simulink model "ev_battery_sim"  (R2026b)
settings: Solver=ode23t  StopTime=60.0  MaxStep=0.05
undefined symbols (not defined in the file or in its folder): Current_A, Temp_C, Voltage_V
libraries: fl_lib x10, nesl_utility x6, EdgeImpulse_Library x2, batteryecm_lib x1
settings Model: Creator=HP  LastModifiedBy=HP
settings SimscapeCC: SimscapeLogType=all  SimscapeNominalValues="[{\"value\":\"1\",\"unit\":\"A\"},{\"value\":\"1\",\"unit\":\"bar\"},{\"value\":\"1\",\"unit\":\"cm^2\"},{\"value\":\"1\",\"unit\":\"cm^3/s\"},{\"value\":\"1\",\"unit\":\"kJ/kg\"},{\"value\":\"1\",\"unit\":\"kW\"},{\"value\":\"1\",\"unit\":\"l\"},{\"value\":\"1\",\"unit\":\"N\"},{\"value\":\"1\",\"unit\":\"N*m\"},{\"value\":\"1\",\"unit\":\"V\"},{\"value\":\"0.001\",\"unit\":\"Wb\"}]"  SimscapeUseEnergyAccounting=off

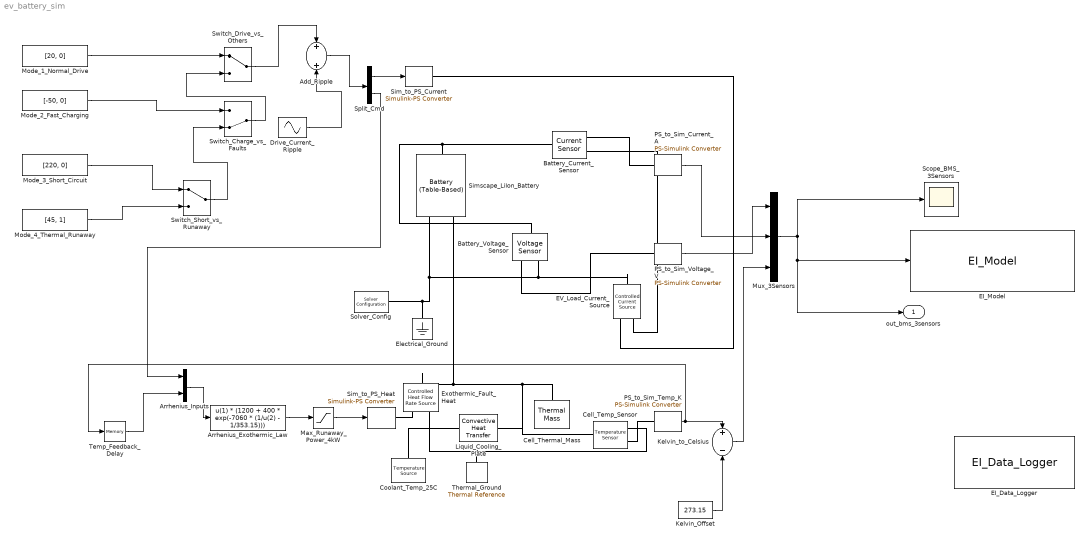
== system ev_battery_sim ==
  Add_Ripple : Sum
  Arrhenius_Exothermic_Law : Fcn  Expr=u(1) * (1200 + 400 * exp(-7060 * (1/u(2) - 1/353.15)))
  Arrhenius_Inputs : Mux  Inputs=2
  Battery_Current_Sensor : fl_lib/Electrical/Electrical Sensors/Current Sensor
  Battery_Voltage_Sensor : fl_lib/Electrical/Electrical Sensors/Voltage Sensor
  Cell_Temp_Sensor : fl_lib/Thermal/Thermal Sensors/Temperature Sensor  temperature_measure=foundation.enum.MeasurementReference.difference
  Cell_Thermal_Mass : fl_lib/Thermal/Thermal Elements/Thermal Mass  mass_type=foundation.enum.constant_variable.constant  mass=0.40 kg  sp_heat=1000 J/(K*kg)  mass_min=1e-6 kg  num_ports=foundation.enum.numPorts2.one  m_specify=off  m_priority=High  m=1 kg  m_nominal_specify=off  m_nominal_value=1  m_nominal_unit=kg  T_specify=on  T_priority=High  T=298.15 K  T_nominal_specify=off  T_nominal_value=1  T_nominal_unit=K  Q_specify=off  Q_priority=None  Q=0 W  Q_nominal_specify=off  Q_nominal_value=1  Q_nominal_unit=W
  Coolant_Temp_25C : fl_lib/Thermal/Thermal Sources/Temperature Source  temperature=298.15 K
  Drive_Current_Ripple : Sin  Amplitude=[2.5, 0]  Frequency=2*pi*0.5  SampleTime=0.05
  EI_Data_Logger : EdgeImpulse_Library/EI_Data_Logger  ei_enabled=on  ei_skip_zero=on  ei_label=Normal_Drive  ei_window_sec=3  ei_max_chunks=0  ei_category=training  ei_sensors=Voltage_V,Current_A,Temp_C  ei_units=V,A,Cel  ei_apikey=ei_bdf74ae27c7bb8ce14bbbb5e7690b771b2b0dc35a7d65027  ei_outdir=default
      settings: SourceProductName=Edge Impulse TinyML
  EI_Model : EdgeImpulse_Library/EI_Model  ei_zip_path=C:\Users\HP\Downloads\bms_system-cpp-mcu-v1-impulse-#1.zip  ei_show_hud=on  ei_verbose=on  ei_step_sec=0.25
      settings: SourceProductName=Edge Impulse TinyML
  EV_Load_Current_Source : fl_lib/Electrical/Electrical Sources/Controlled Current Source
  Electrical_Ground : fl_lib/Electrical/Electrical Elements/Electrical Reference
  Exothermic_Fault_Heat : fl_lib/Thermal/Thermal Sources/Controlled Heat Flow Rate Source
  Kelvin_Offset : Constant  Value=273.15
  Kelvin_to_Celsius : Sum  Inputs=+-
  Liquid_Cooling_Plate : fl_lib/Thermal/Thermal Elements/Convective Heat Transfer  thermal_type=foundation.enum.constant_variable.constant  area=0.02 m^2  heat_tr_coeff=200 W/(K*m^2)  min_heat_tr_coeff=1e-3 W/(K*m^2)  T_specify=off  T_priority=None  T=0 K  T_nominal_specify=off  T_nominal_value=1  T_nominal_unit=K  Q_specify=off  Q_priority=None  Q=0 W  Q_nominal_specify=off  Q_nominal_value=1  Q_nominal_unit=W
  Max_Runaway_Power_4kW : Saturate  UpperLimit=4000  LowerLimit=0
  Mode_1_Normal_Drive : Constant  Value=[20, 0]
  Mode_2_Fast_Charging : Constant  Value=[-50, 0]
  Mode_3_Short_Circuit : Constant  Value=[220, 0]
  Mode_4_Thermal_Runaway : Constant  Value=[45, 1]
  Mux_3Sensors : Mux  Inputs=3
  PS_to_Sim_Current_A : nesl_utility/PS-Simulink Converter  PhysicalDomain=network_engine_domain  SubClassName=ps_output  LeftPortType=input  RightPortType=output  PseudoPeriodic=off  Frequencies=[]  VectorFormat=inherit  Unit=inherit  AffineConversion=off
  PS_to_Sim_Temp_K : nesl_utility/PS-Simulink Converter  PhysicalDomain=network_engine_domain  SubClassName=ps_output  LeftPortType=input  RightPortType=output  PseudoPeriodic=off  Frequencies=[]  VectorFormat=inherit  Unit=inherit  AffineConversion=off
  PS_to_Sim_Voltage_V : nesl_utility/PS-Simulink Converter  PhysicalDomain=network_engine_domain  SubClassName=ps_output  LeftPortType=input  RightPortType=output  PseudoPeriodic=off  Frequencies=[]  VectorFormat=inherit  Unit=inherit  AffineConversion=off
  Scope_BMS_3Sensors : Scope
  Sim_to_PS_Current : nesl_utility/Simulink-PS Converter  PhysicalDomain=network_engine_domain  SubClassName=ps_input  LeftPortType=input  RightPortType=output  PseudoPeriodic=off  Frequencies=[]  NoiseDistribution=none  NoiseParameters=[]  Unit=1  AffineConversion=off  FilteringAndDerivatives=provide  SimscapeFilterOrder=1  InputFilterTimeConstant=0.001  UdotUserProvided=0
  Sim_to_PS_Heat : nesl_utility/Simulink-PS Converter  PhysicalDomain=network_engine_domain  SubClassName=ps_input  LeftPortType=input  RightPortType=output  PseudoPeriodic=off  Frequencies=[]  NoiseDistribution=none  NoiseParameters=[]  Unit=1  AffineConversion=off  FilteringAndDerivatives=provide  SimscapeFilterOrder=1  InputFilterTimeConstant=0.001  UdotUserProvided=0
  Simscape_LiIon_Battery : batteryecm_lib/Battery (Table-Based)  SOC_vec=[0, .1, .25, .5, .75, .9, 1]  T_dependence=simscape.enum.tablebattery.temperature_dependence.yes  prm_dir=simscape.enum.tablebattery.prm_dir.noCurrentDirectionality  T_vec=[278, 293, 313] K  V0_mat=[3.49, 3.5, 3.51; 3.55, 3.57, 3.56; 3.62, 3.63, 3.64; 3.71, 3.71, 3.72; 3.91, 3.93, 3.94; 4.07, 4.08, 4.08; 4.19, 4.19, 4.19] V  V0_vec=[3.5057, 3.566, 3.6337, 3.7127, 3.9259, 4.0777, 4.1928] V  V_range=[0, inf] V  R0_mat=[.0117, .0085, .009; .011, .0085, .009; .0114, .0087, .0092; .0107, .0082, .0088; .0107, .0083, .0091; .0113, .0085, .0089; .0116, .0085, .0089] Ohm  R0_vec=[.0085, .0085, .0087, .0082, .0083, .0085, .0085] Ohm  R0_dis_mat=[.0117, .0085, .009; .011, .0085, .009; .0114, .0087, .0092; .0107, .0082, .0088; .0107, .0083, .0091; .0113, .0085, .0089; .0116, .0085, .0089] Ohm  R0_dis_vec=[.0085, .0085, .0087, .0082, .0083, .0085, .0085] Ohm  R0_ch_mat=[.0117, .0085, .009; .011, .0085, .009; .0114, .0087, .0092; .0107, .0082, .0088; .0107, .0083, .0091; .0113, .0085, .0089; .0116, .0085, .0089] Ohm  R0_ch_vec=[.0085, .0085, .0087, .0082, .0083, .0085, .0085] Ohm  AH=27 A*hr  prm_leak=simscape.enum.tablebattery.prm_leak.disabled  Rleak_vec=[8000, 7000, 6000] Ohm  Rleak=7e3 Ohm  extrapolation_option=simscape.enum.extrapolation.nearest  SOC_port=simscape.enum.tablebattery.enable.no  prm_dyn=simscape.enum.tablebattery.prm_dyn.off  R1_mat=[.0109, .0029, .0013; .0069, .0024, .0012; .0047, .0026, .0013; .0034, .0016, .001; .0033, .0023, .0014; .0033, .0018, .0011; .0028, .0017, .0011] Ohm  R1_vec=[.0029, .0024, .0026, .0016, .0023, .0018, .0017] Ohm  tau1_mat=[20, 36, 39; 31, 45, 39; 109, 105, 61; 36, 29, 26; 59, 77, 67; 40, 33, 29; 25, 39, 33] s  tau1_vec=[36, 45, 105, 29, 77, 33, 39] s  R2_mat=[.0109, .0029, .0013; .0069, .0024, .0012; .0047, .0026, .0013; .0034, .0016, .001; .0033, .0023, .0014; .0033, .0018, .0011; .0028, .0017, .0011] Ohm  R2_vec=[.0029, .0024, .0026, .0016, .0023, .0018, .0017] Ohm  tau2_mat=[20, 36, 39; 31, 45, 39; 109, 105, 61; 36, 29, 26; 59, 77, 67; 40, 33, 29; 25, 39, 33] s  tau2_vec=[36, 45, 105, 29, 77, 33, 39] s  R3_mat=[.0109, .0029, .0013; .0069, .0024, .0012; .0047, .0026, .0013; .0034, .0016, .001; .0033, .0023, .0014; .0033, .0018, .0011; .0028, .0017, .0011] Ohm  R3_vec=[.0029, .0024, .0026, .0016, .0023, .0018, .0017] Ohm  tau3_mat=[20, 36, 39; 31, 45, 39; 109, 105, 61; 36, 29, 26; 59, 77, 67; 40, 33, 29; 25, 39, 33] s  tau3_vec=[36, 45, 105, 29, 77, 33, 39] s  R4_mat=[.0109, .0029, .0013; .0069, .0024, .0012; .0047, .0026, .0013; .0034, .0016, .001; .0033, .0023, .0014; .0033, .0018, .0011; .0028, .0017, .0011] Ohm  R4_vec=[.0029, .0024, .0026, .0016, .0023, .0018, .0017] Ohm  tau4_mat=[20, 36, 39; 31, 45, 39; 109, 105, 61; 36, 29, 26; 59, 77, 67; 40, 33, 29; 25, 39, 33] s  tau4_vec=[36, 45, 105, 29, 77, 33, 39] s  R5_mat=[.0109, .0029, .0013; .0069, .0024, .0012; .0047, .0026, .0013; .0034, .0016, .001; .0033, .0023, .0014; .0033, .0018, .0011; .0028, .0017, .0011] Ohm  R5_vec=[.0029, .0024, .0026, .0016, .0023, .0018, .0017] Ohm  tau5_mat=[20, 36, 39; 31, 45, 39; 109, 105, 61; 36, 29, 26; 59, 77, 67; 40, 33, 29; 25, 39, 33] s  tau5_vec=[36, 45, 105, 29, 77, 33, 39] s  prm_fade=simscape.enum.tablebattery.prm_fade.disabled  N0=100  dV0=0  dR0=0  dAH=0  dRleak=0  dR1=0  dR2=0  dR3=0  dR4=0  dR5=0  N0vec=[0, 100, 200, 300]  Tfadevec=[298.15, 323.15] K  dV0vec=[0, 0, 0, 0]  dR0vec=[0, 0, 0, 0]  dAHvec=[0, 0, 0, 0]  dRleakvec=[0, 0, 0, 0]  dR1vec=[0, 0, 0, 0]  dR2vec=[0, 0, 0, 0]  dR3vec=[0, 0, 0, 0]  dR4vec=[0, 0, 0, 0]  dR5vec=[0, 0, 0, 0]  dV0mat=[0, 0; 0, 0; 0, 0; 0, 0]  dR0mat=[0, 0; 0, 0; 0, 0; 0, 0]  dAHmat=[0, 0; 0, 0; 0, 0; 0, 0]  dRleakmat=[0, 0; 0, 0; 0, 0; 0, 0]  dR1mat=[0, 0; 0, 0; 0, 0; 0, 0]  dR2mat=[0, 0; 0, 0; 0, 0; 0, 0]  dR3mat=[0, 0; 0, 0; 0, 0; 0, 0]  dR4mat=[0, 0; 0, 0; 0, 0; 0, 0]  dR5mat=[0, 0; 0, 0; 0, 0; 0, 0]  prm_age_modeling=simscape.enum.tablebattery.prm_age_modeling.equation  storage_dt_age_vec=[0] d  storage_T_age_vec=[273] K  prm_age_OCV=simscape.enum.tablebattery.prm_age_OCV.OCV  OCV_age=0.9  SOC_age=0.6  prm_age_resistance=simscape.enum.tablebattery.prm_age.disabled  OCV_scaling_age_resistance=2.2134e6  OCV_offset_age_resistance=1.632e6  temp_exp_age_resistance=0.515833569 V  t_exp_age_resistance=0.75  T_age_vec_resistance=[273.15, 298.15, 323.15] K  dt_age_vec_resistance=[0, 90, 180, 270] d  dR0_age_vec=[0, 0, 0]  t_meas_dR0_age=100 d  dR0_age_mat=[0, 0, 0; 0, 0, 0; 0, 0, 0; 0, 0, 0]  prm_age_capacity=simscape.enum.tablebattery.prm_age.disabled  OCV_scaling_age_capacity=1.5097e07  OCV_offset_age_capacity=8.3625e06  temp_exp_age_capacity=0.6011 V  t_exp_age_capacity=0.75  T_age_vec_capacity=[273.15, 298.15, 323.15] K  dt_age_vec_capacity=[0, 90, 180, 270] d  dAH_age_vec=[0, 0, 0]  t_meas_dAH_age=100 d  dAH_age_mat=[0, 0, 0; 0, 0, 0; 0, 0, 0; 0, 0, 0]  thermal_port=1  temperature=298.15 K  thermal_mass=100 J/K  i_specify=off  i_priority=None  i=0 A  i_nominal_specify=off  i_nominal_value=1  i_nominal_unit=A  v_specify=off  v_priority=None  v=0 V  v_nominal_specify=off  v_nominal_value=1  v_nominal_unit=V  stateOfCharge_specify=on  stateOfCharge_priority=High  stateOfCharge=0.9  stateOfCharge_nominal_specify=off  stateOfCharge_nominal_value=1  stateOfCharge_nominal_unit=1  num_cycles_specify=off  num_cycles_priority=High  num_cycles=0  num_cycles_nominal_specify=off  num_cycles_nominal_value=1  num_cycles_nominal_unit=1  cell_temperature_specify=off  cell_temperature_priority=High  cell_temperature=298.15 K  cell_temperature_nominal_specify=off  cell_temperature_nominal_value=1  cell_temperature_nominal_unit=K
  Solver_Config : nesl_utility/Solver Configuration  PhysicalDomain=network_engine_domain  SubClassName=solver  LeftPortType=input  RightPortType=generic  Tones=[]  Harmonics=[]  SimulateNoise=off  Profile=off  UseLocalSampling=off  EnableSwitchedLinearOptims=on  FrequencyDomain=off  UseCCode=off  RelTol=0.001  AbsTol=0.001  MinStep=1e-09  ToWorkspace=off  RevertToSquareIcSolve=off  NumHomotopyIterations=100  PhasorMode=off  PhasorModeNumHarmonics=1  ConsistencySolver=NEWTON_XTOL_AFTER_FTOL  CanonicalOrdering=CANONICAL  OptimizeIntermediates=OPTIMIZED  MulticoreSolverChoice=BACKWARD_EULER  IndexReductionMethod=DerivativeReplacement  DoDC=off  ResidualTolerance=1e-09  ConsistencyTolSource=GLOBAL  ConsistencyAbsTol=0.001  ConsistencyRelTol=0.001  ConsistencyTolFactor=0.001  UseLocalSolver=off  LocalSolverChoice=NE_BACKWARD_EULER_ADVANCER  ResolveIndetEquations=on  FunctionEvalNumThread=1  LocalSolverSampleTime=0.001  DoFixedCost=off  MaxNonlinIter=3  MaxModeIter=2  ComputeImpulses=off  ImpulseIterations=2  LinearAlgebra=auto  LinearAlgebraNumThread=0  EquationFormulation=NE_TIME_EF  DelaysMemoryBudget=1024  AutomaticFiltering=on  FilteringTimeConstant=0.001  PartitionStorageMethod=AS_NEEDED  PartitionMemoryBudget=1024  PartitionMethod=BALANCED  MultibodyUseLocalSolver=off  MultibodyLocalSolverChoice=ODE1  MultibodyLocalSolverSampleTime=0.001
  Split_Cmd : Demux  Outputs=2
  Switch_Charge_vs_Faults : ManualSwitch  CurrentSetting=0
  Switch_Drive_vs_Others : ManualSwitch
  Switch_Short_vs_Runaway : ManualSwitch
  Temp_Feedback_Delay : Memory  InitialCondition=298.15
  Thermal_Ground : fl_lib/Thermal/Thermal Elements/Thermal Reference
  out_bms_3sensors : Outport
  wires:
  Mode_3_Short_Circuit/1 -> Switch_Short_vs_Runaway/1
  Mode_4_Thermal_Runaway/1 -> Switch_Short_vs_Runaway/2
  Mode_2_Fast_Charging/1 -> Switch_Charge_vs_Faults/1
  Switch_Short_vs_Runaway/1 -> Switch_Charge_vs_Faults/2
  Mode_1_Normal_Drive/1 -> Switch_Drive_vs_Others/1
  Switch_Charge_vs_Faults/1 -> Switch_Drive_vs_Others/2
  Switch_Drive_vs_Others/1 -> Add_Ripple/1
  Drive_Current_Ripple/1 -> Add_Ripple/2
  Add_Ripple/1 -> Split_Cmd/1
  Split_Cmd/1 -> Sim_to_PS_Current/1
  Arrhenius_Inputs/1 -> Arrhenius_Exothermic_Law/1
  Arrhenius_Exothermic_Law/1 -> Max_Runaway_Power_4kW/1
  Max_Runaway_Power_4kW/1 -> Sim_to_PS_Heat/1
  PS_to_Sim_Temp_K/1 -> Temp_Feedback_Delay/1, Kelvin_to_Celsius/1
  Temp_Feedback_Delay/1 -> Arrhenius_Inputs/2
  Kelvin_Offset/1 -> Kelvin_to_Celsius/2
  PS_to_Sim_Voltage_V/1 -> Mux_3Sensors/1
  PS_to_Sim_Current_A/1 -> Mux_3Sensors/2
  Kelvin_to_Celsius/1 -> Mux_3Sensors/3
  Mux_3Sensors/1 -> EI_Model/1, out_bms_3sensors/1, Scope_BMS_3Sensors/1
  Split_Cmd/2 -> Arrhenius_Inputs/1
  connections:
  Sim_to_PS_Current/RConn1 -- EV_Load_Current_Source/RConn1
  Simscape_LiIon_Battery/LConn1 -- Battery_Current_Sensor/LConn1 -- Battery_Voltage_Sensor/LConn1
  Battery_Current_Sensor/RConn2 -- EV_Load_Current_Source/RConn2
  EV_Load_Current_Source/LConn1 -- Simscape_LiIon_Battery/RConn1 -- Solver_Config/RConn1 -- Electrical_Ground/LConn1 -- Battery_Voltage_Sensor/RConn2
  Sim_to_PS_Heat/RConn1 -- Exothermic_Fault_Heat/RConn1
  Simscape_LiIon_Battery/RConn2 -- Exothermic_Fault_Heat/LConn1 -- Liquid_Cooling_Plate/RConn1 -- Cell_Temp_Sensor/LConn1 -- Cell_Thermal_Mass/LConn1
  Thermal_Ground/LConn1 -- Exothermic_Fault_Heat/RConn2 -- Cell_Temp_Sensor/RConn1
  Coolant_Temp_25C/LConn1 -- Liquid_Cooling_Plate/LConn1
  Battery_Voltage_Sensor/RConn1 -- PS_to_Sim_Voltage_V/LConn1
  Battery_Current_Sensor/RConn1 -- PS_to_Sim_Current_A/LConn1
  Cell_Temp_Sensor/RConn2 -- PS_to_Sim_Temp_K/LConn1
